simulink model "A_ZH_Z3"  (R2026a)
settings: Solver=VariableStepAuto  StopTime=2  MaxStep=0.1/25
settings Model: Creator=Szalay  LastModifiedBy=Szalay

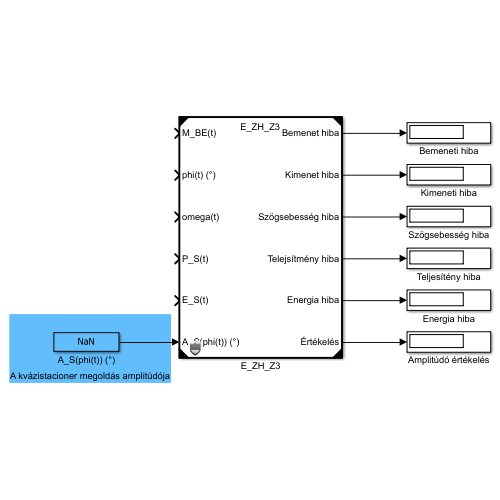
[thumbnail: Simulink's stored preview of the top-level diagram]
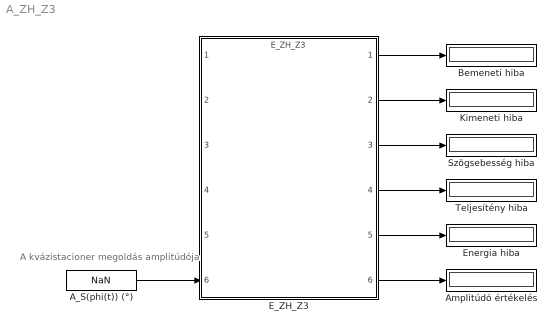
== system A_ZH_Z3 ==
  note: A kvázistacioner megoldás amplitúdója
  A_S(phi(t)) (°) : Constant  Value=NaN
  Amplitúdó értékelés : Display
  Bemeneti hiba : Display
  E_ZH_Z3 : ModelReference  ModelNameDialog=E_ZH_Z3.slxp  ModelReferenceVersion=3.4  CopyOfModelProtected=on
  Energia hiba : Display
  Kimeneti hiba : Display
  Szögsebesség hiba : Display
  Teljesítény hiba : Display
  wires:
  E_ZH_Z3/1 -> Bemeneti hiba/1
  E_ZH_Z3/2 -> Kimeneti hiba/1
  A_S(phi(t)) (°)/1 -> E_ZH_Z3/6
  E_ZH_Z3/3 -> Szögsebesség hiba/1
  E_ZH_Z3/4 -> Teljesítény hiba/1
  E_ZH_Z3/5 -> Energia hiba/1
  E_ZH_Z3/6 -> Amplitúdó értékelés/1
